simulink model "W09_E3_DelayMargin"  (R2024b)
settings: Solver=ode45  StartTime=0.0  StopTime=t_end  MaxStep=0.02  RelTol=1e-3
PreLoadFcn:
  | % W09_E3_DelayMargin 기본 파라미터 (모델을 열 때 자동 실행)
  | defs = { 'K',0.5 ; 'tau_d',0 ; 't_end',80 ;
  |          'numG',1 ; 'denG',[1 2 1 0] };
  | for ii = 1:size(defs,1)
  |     if ~evalin('base', sprintf('exist(''%s'',''var'')', defs{ii,1}))
  |         assignin('base', defs{ii,1}, defs{ii,2});
  |     end
  | end
  | clear defs ii
values from neighbouring files (symbols this model uses):
  K = 0.5    [W09_02_pm_to_time.m]    (also in W09_03_run_simulink.m; W09_07_examples.m)
  tau_d = tau_list(i)    [W09_03_run_simulink.m]    (also in W09_07_examples.m)
undefined symbols (not defined in the file or in its folder): denG, numG
settings Model: Creator=admin  LastModifiedBy=admin

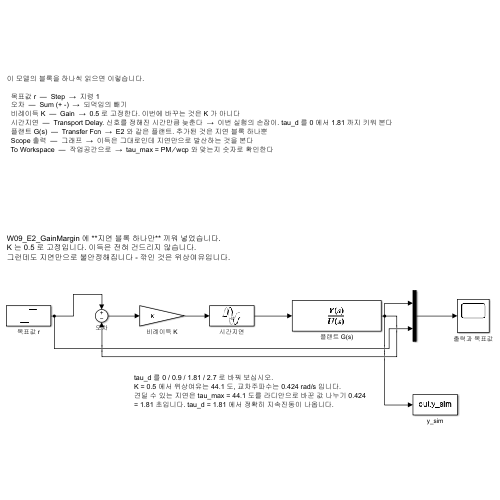
[thumbnail: Simulink's stored preview of the top-level diagram]
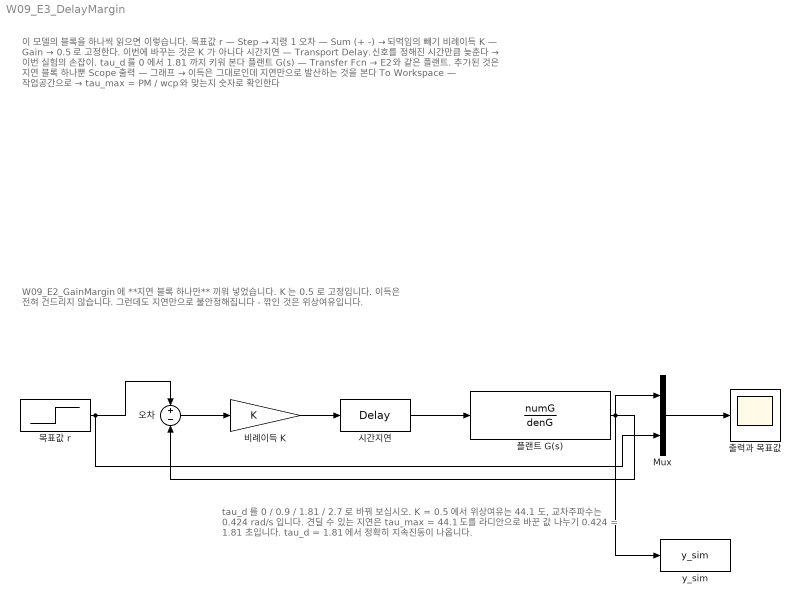
== system W09_E3_DelayMargin ==
  note: W09_E2_GainMargin 에 **지연 블록 하나만** 끼워 넣었습니다.
      | K 는 0.5 로 고정입니다. 이득은 전혀 건드리지 않습니다.
      | 그런데도 지연만으로 불안정해집니다 - 깎인 것은 위상여유입니다.
  note: tau_d 를 0 / 0.9 / 1.81 / 2.7 로 바꿔 보십시오.
      | K = 0.5 에서 위상여유는 44.1 도, 교차주파수는 0.424 rad/s 입니다.
      | 견딜 수 있는 지연은 tau_max = 44.1 도를 라디안으로 바꾼 값 나누기 0.424
      | = 1.81 초입니다. tau_d = 1.81 에서 정확히 지속진동이 나옵니다.
  note: 이 모델의 블록을 하나씩 읽으면 이렇습니다.
      |
      |   목표값 r  —  Step  →  지령 1
      |   오차  —  Sum (+ -)  →  되먹임의 빼기
      |   비례이득 K  —  Gain  →  0.5 로 고정한다. 이번에 바꾸는 것은 K 가 아니다
      |   시간지연  —  Transport Delay. 신호를 정해진 시간만큼 늦춘다  →  이번 실험의 손잡이. tau_d 를 0 에서 1.81 까지 키워 본다
      |   플랜트 G(s)  —  Transfer Fcn  →  E2 와 같은 플랜트. 추가된 것은 지연 블록 하나뿐
      |   Scope 출력  —  그래프  →  이득은 그대로인데 지연만으로 발산하는 것을 본다
      |   To Workspace  —  작업공간으로  →  tau_max = PM ∕ wcp 와 맞는지 숫자로 확인한다
  Mux : Mux  Inputs=2
  y_sim : ToWorkspace  VariableName=y_sim  SaveFormat=Timeseries  SampleTime=-1
  목표값 r : Step  Time=0  SampleTime=0
  비례이득 K : Gain  Gain=K
  시간지연 : TransportDelay  DelayTime=tau_d
  오차 : Sum  Inputs=+-
  출력과 목표값 : Scope
  플랜트 G(s) : TransferFcn  Numerator=numG  Denominator=denG
  wires:
  목표값 r/1 -> 오차/1, Mux/2
  오차/1 -> 비례이득 K/1
  비례이득 K/1 -> 시간지연/1
  시간지연/1 -> 플랜트 G(s)/1
  플랜트 G(s)/1 -> 오차/2, Mux/1, y_sim/1
  Mux/1 -> 출력과 목표값/1
